simulink model "model_7dof&14dof"  (R2023b)
settings: Solver=FixedStepAuto  StartTime=0.0  StopTime=25  FixedStep=0.01  RelTol=1e-3  EnableMultiTasking=on
values from neighbouring files (symbols this model uses):
  A = 5    [unlinear_vehicle_Parameters.m]
  Bf = 1.725    [unlinear_vehicle_Parameters.m]
  Br = 1.750    (= 1.75)    [unlinear_vehicle_Parameters.m]
  Cd = 0.4    [unlinear_vehicle_Parameters.m]
  Cs_f = 4302    [unlinear_vehicle_Parameters.m]
  f = 0.01    [unlinear_vehicle_Parameters.m]
  g = 9.8    [Truck_simulate.m]    (also in unlinear_vehicle_Parameters.m)
  He = 0.45    [unlinear_vehicle_Parameters.m]
  hg = 0.781    [unlinear_vehicle_Parameters.m]
  Hp = 0.2    [unlinear_vehicle_Parameters.m]
  I_tire = 0.7    [unlinear_vehicle_Parameters.m]
  Ix = 423.3    [unlinear_vehicle_Parameters.m]
  Iy = 1762.5    [unlinear_vehicle_Parameters.m]
  Iz = 1762.5    [unlinear_vehicle_Parameters.m]
  ks_f = 189000    [unlinear_vehicle_Parameters.m]
  kw = 220000    [unlinear_vehicle_Parameters.m]
  L = 3.140    (= 3.14)    [unlinear_vehicle_Parameters.m]
  Lf = 1.330    (= 1.33)    [unlinear_vehicle_Parameters.m]
  Lr = 3.140 - 1.330    (= 1.81)    [unlinear_vehicle_Parameters.m]
  m = m_sprung + m_load + m_unsprung    (= 10505)    [Truck_simulate.m]    (also in unlinear_vehicle_Parameters.m = 1407.3)
  mb = 1128.5 + 000    (= 1128.5)    [unlinear_vehicle_Parameters.m]
  mw = 139.4 / 2    (= 69.7)    [unlinear_vehicle_Parameters.m]
  p = 1.206    [unlinear_vehicle_Parameters.m]
  r = 0.510    (= 0.51)    [Truck_simulate.m]    (also in unlinear_vehicle_Parameters.m = 0.287)
  vx0 = 5    [Truck_simulate.m]    (also in unlinear_vehicle_Parameters.m)
  vy0 = 0    [Truck_simulate.m]    (also in unlinear_vehicle_Parameters.m)
  w0 = vx0 / r    (= 9.80392156863)    [Truck_simulate.m]    (also in unlinear_vehicle_Parameters.m = 17.4216027875)
  wz0 = 0    [Truck_simulate.m]    (also in unlinear_vehicle_Parameters.m)
(part 2 of 2)

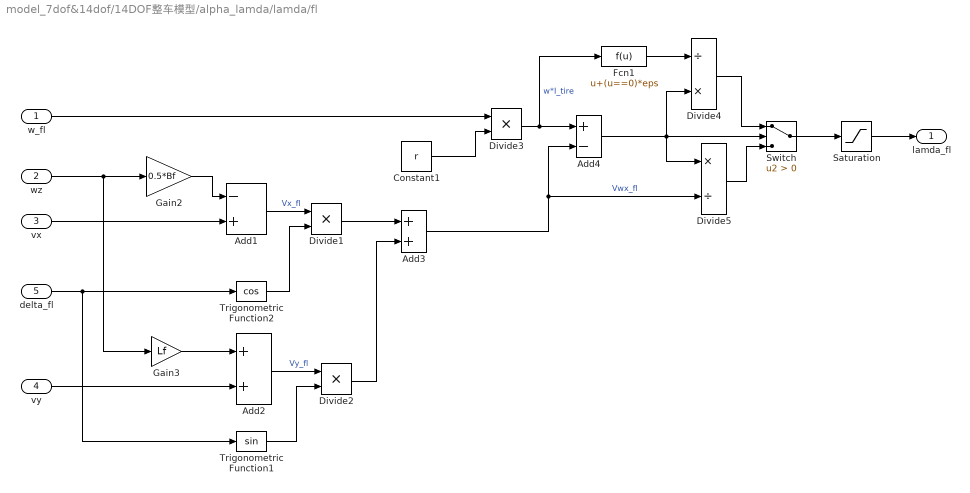
== system model_7dof&14dof/14DOF整车模型/alpha_lamda/lamda/fl ==
  w_fl : Inport
  wz : Inport  Port=2
  vx : Inport  Port=3
  vy : Inport  Port=4
  delta_fl : Inport  Port=5
  Add1 : Sum  Inputs=-+
  Add2 : Sum
  Add3 : Sum
  Add4 : Sum  Inputs=+-
  Constant1 : Constant  Value=r
  Divide1 : Product  Inputs=**
  Divide2 : Product  Inputs=**
  Divide3 : Product  Inputs=**
  Divide4 : Product  Inputs=/*
  Divide5 : Product  Inputs=*/
  Fcn1 : Fcn  Expr=u+(u==0)*eps
  Gain2 : Gain  Gain=0.5*Bf
  Gain3 : Gain  Gain=Lf
  Saturation : Saturate  UpperLimit=1  LowerLimit=-1
  Switch : Switch  Criteria=u2 > Threshold  SaturateOnIntegerOverflow=off  InputSameDT=off
  Trigonometric Function1 : Trigonometry
  Trigonometric Function2 : Trigonometry  Operator=cos
  lamda_fl : Outport
  wires:
  Saturation/1 -> lamda_fl/1
  Divide3/1 -> Fcn1/1, Add4/1  "w*I_tire"
  Constant1/1 -> Divide3/2
  w_fl/1 -> Divide3/1
  Divide2/1 -> Add3/2
  Divide1/1 -> Add3/1
  Trigonometric Function1/1 -> Divide2/2
  Add2/1 -> Divide2/1  "Vy_fl"
  Gain3/1 -> Add2/1
  vy/1 -> Add2/2
  Trigonometric Function2/1 -> Divide1/2
  delta_fl/1 -> Trigonometric Function1/1, Trigonometric Function2/1
  Add1/1 -> Divide1/1  "Vx_fl"
  wz/1 -> Gain2/1, Gain3/1
  Gain2/1 -> Add1/1
  vx/1 -> Add1/2
  Fcn1/1 -> Divide4/1
  Divide5/1 -> Switch/3
  Divide4/1 -> Switch/1
  Add4/1 -> Divide5/1, Divide4/2, Switch/2
  Add3/1 -> Divide5/2, Add4/2  "Vwx_fl"
  Switch/1 -> Saturation/1

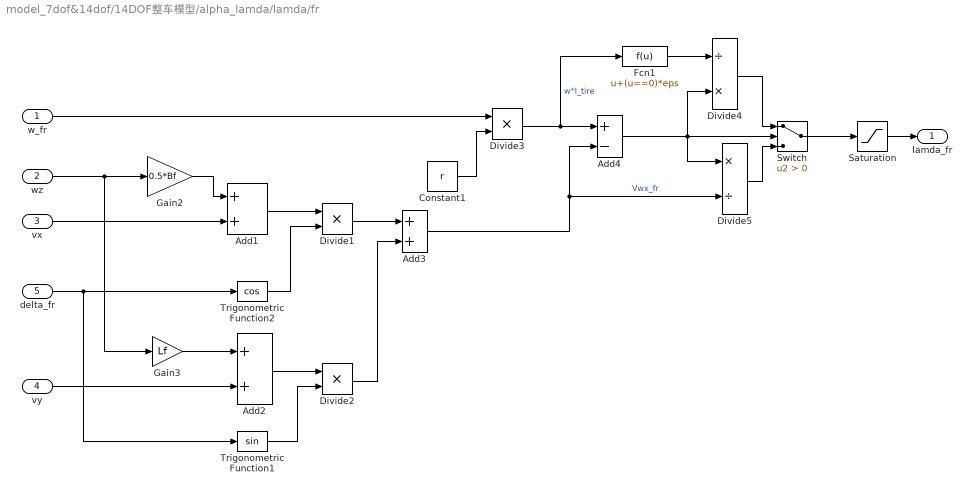
== system model_7dof&14dof/14DOF整车模型/alpha_lamda/lamda/fr ==
  w_fr : Inport
  wz : Inport  Port=2
  vx : Inport  Port=3
  vy : Inport  Port=4
  delta_fr : Inport  Port=5
  Add1 : Sum
  Add2 : Sum
  Add3 : Sum
  Add4 : Sum  Inputs=+-
  Constant1 : Constant  Value=r
  Divide1 : Product  Inputs=**
  Divide2 : Product  Inputs=**
  Divide3 : Product  Inputs=**
  Divide4 : Product  Inputs=/*
  Divide5 : Product  Inputs=*/
  Fcn1 : Fcn  Expr=u+(u==0)*eps
  Gain2 : Gain  Gain=0.5*Bf
  Gain3 : Gain  Gain=Lf
  Saturation : Saturate  UpperLimit=1  LowerLimit=-1
  Switch : Switch  Criteria=u2 > Threshold  SaturateOnIntegerOverflow=off  InputSameDT=off
  Trigonometric Function1 : Trigonometry
  Trigonometric Function2 : Trigonometry  Operator=cos
  lamda_fr : Outport
  wires:
  Switch/1 -> Saturation/1
  Add3/1 -> Add4/2, Divide5/2  "Vwx_fr"
  Add4/1 -> Switch/2, Divide4/2, Divide5/1
  Divide4/1 -> Switch/1
  Divide5/1 -> Switch/3
  Fcn1/1 -> Divide4/1
  Divide3/1 -> Add4/1, Fcn1/1  "w*I_tire"
  Constant1/1 -> Divide3/2
  w_fr/1 -> Divide3/1
  Divide2/1 -> Add3/2
  Divide1/1 -> Add3/1
  Trigonometric Function1/1 -> Divide2/2
  Add2/1 -> Divide2/1
  Gain3/1 -> Add2/1
  vy/1 -> Add2/2
  Trigonometric Function2/1 -> Divide1/2
  delta_fr/1 -> Trigonometric Function1/1, Trigonometric Function2/1
  Add1/1 -> Divide1/1
  wz/1 -> Gain2/1, Gain3/1
  Gain2/1 -> Add1/1
  vx/1 -> Add1/2
  Saturation/1 -> lamda_fr/1

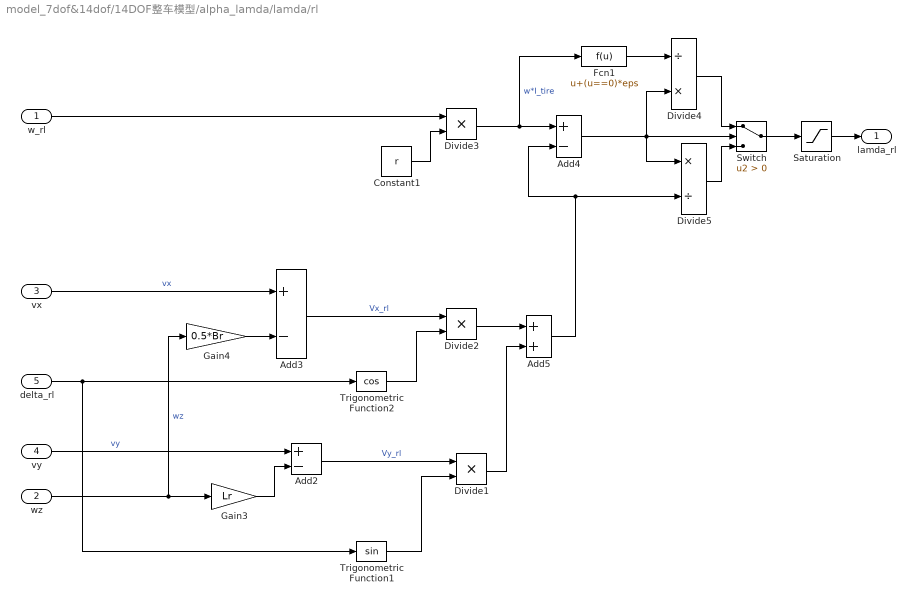
== system model_7dof&14dof/14DOF整车模型/alpha_lamda/lamda/rl ==
  w_rl : Inport
  wz : Inport  Port=2
  vx : Inport  Port=3
  vy : Inport  Port=4
  delta_rl : Inport  Port=5
  Add2 : Sum  Inputs=+-
  Add3 : Sum  Inputs=+-
  Add4 : Sum  Inputs=+-
  Add5 : Sum
  Constant1 : Constant  Value=r
  Divide1 : Product  Inputs=**
  Divide2 : Product  Inputs=**
  Divide3 : Product  Inputs=**
  Divide4 : Product  Inputs=/*
  Divide5 : Product  Inputs=*/
  Fcn1 : Fcn  Expr=u+(u==0)*eps
  Gain3 : Gain  Gain=Lr
  Gain4 : Gain  Gain=0.5*Br
  Saturation : Saturate  UpperLimit=1  LowerLimit=-1
  Switch : Switch  Criteria=u2 > Threshold  SaturateOnIntegerOverflow=off  InputSameDT=off
  Trigonometric Function1 : Trigonometry
  Trigonometric Function2 : Trigonometry  Operator=cos
  lamda_rl : Outport
  wires:
  Switch/1 -> Saturation/1
  Add4/1 -> Switch/2, Divide4/2, Divide5/1
  Divide4/1 -> Switch/1
  Divide5/1 -> Switch/3
  Fcn1/1 -> Divide4/1
  Divide3/1 -> Add4/1, Fcn1/1  "w*I_tire"
  Constant1/1 -> Divide3/2
  w_rl/1 -> Divide3/1
  Saturation/1 -> lamda_rl/1
  Gain4/1 -> Add3/2
  wz/1 -> Gain3/1, Gain4/1  "wz"
  vy/1 -> Add2/1  "vy"
  vx/1 -> Add3/1  "vx"
  Add3/1 -> Divide2/1  "Vx_rl"
  Add2/1 -> Divide1/1  "Vy_rl"
  Gain3/1 -> Add2/2
  delta_rl/1 -> Trigonometric Function1/1, Trigonometric Function2/1
  Trigonometric Function2/1 -> Divide2/2
  Divide2/1 -> Add5/1
  Trigonometric Function1/1 -> Divide1/2
  Divide1/1 -> Add5/2
  Add5/1 -> Add4/2, Divide5/2

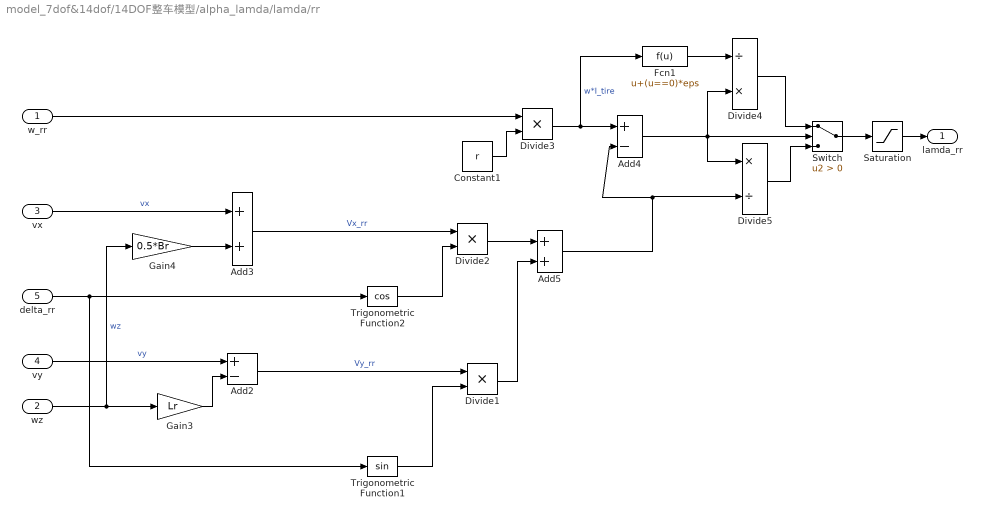
== system model_7dof&14dof/14DOF整车模型/alpha_lamda/lamda/rr ==
  w_rr : Inport
  wz : Inport  Port=2
  vx : Inport  Port=3
  vy : Inport  Port=4
  delta_rr : Inport  Port=5
  Add2 : Sum  Inputs=+-
  Add3 : Sum
  Add4 : Sum  Inputs=+-
  Add5 : Sum
  Constant1 : Constant  Value=r
  Divide1 : Product  Inputs=**
  Divide2 : Product  Inputs=**
  Divide3 : Product  Inputs=**
  Divide4 : Product  Inputs=/*
  Divide5 : Product  Inputs=*/
  Fcn1 : Fcn  Expr=u+(u==0)*eps
  Gain3 : Gain  Gain=Lr
  Gain4 : Gain  Gain=0.5*Br
  Saturation : Saturate  UpperLimit=1  LowerLimit=-1
  Switch : Switch  Criteria=u2 > Threshold  SaturateOnIntegerOverflow=off  InputSameDT=off
  Trigonometric Function1 : Trigonometry
  Trigonometric Function2 : Trigonometry  Operator=cos
  lamda_rr : Outport
  wires:
  Add4/1 -> Switch/2, Divide4/2, Divide5/1
  Divide4/1 -> Switch/1
  Divide5/1 -> Switch/3
  Fcn1/1 -> Divide4/1
  Divide3/1 -> Add4/1, Fcn1/1  "w*I_tire"
  w_rr/1 -> Divide3/1
  Constant1/1 -> Divide3/2
  Switch/1 -> Saturation/1
  Saturation/1 -> lamda_rr/1
  Gain4/1 -> Add3/2
  Gain3/1 -> Add2/2
  Add2/1 -> Divide1/1  "Vy_rr"
  Add3/1 -> Divide2/1  "Vx_rr"
  vx/1 -> Add3/1  "vx"
  vy/1 -> Add2/1  "vy"
  wz/1 -> Gain4/1, Gain3/1  "wz"
  Trigonometric Function2/1 -> Divide2/2
  Divide2/1 -> Add5/1
  Trigonometric Function1/1 -> Divide1/2
  Divide1/1 -> Add5/2
  delta_rr/1 -> Trigonometric Function1/1, Trigonometric Function2/1
  Add5/1 -> Add4/2, Divide5/2

== system model_7dof&14dof/7DOF整车模型/alpha_lamda/alpha/fl ==
  vx : Inport
  vy : Inport  Port=2
  wz : Inport  Port=3
  delta_fl : Inport  Port=4
  Add2 : Sum
  Add3 : Sum  Inputs=+-
  Add4 : Sum  Inputs=-+
  Divide : Product  Inputs=/*
  Gain3 : Gain  Gain=Lf
  Gain4 : Gain  Gain=0.5*Bf
  Trigonometric Function : Trigonometry  Operator=atan
  alpha_fl : Outport
  wires:
  wz/1 -> Gain3/1, Gain4/1
  Add4/1 -> alpha_fl/1
  vy/1 -> Add2/1
  delta_fl/1 -> Add4/2
  vx/1 -> Add3/1
  Trigonometric Function/1 -> Add4/1
  Divide/1 -> Trigonometric Function/1
  Add3/1 -> Divide/1
  Add2/1 -> Divide/2
  Gain4/1 -> Add3/2
  Gain3/1 -> Add2/2

== system model_7dof&14dof/7DOF整车模型/alpha_lamda/alpha/fr ==
  vx : Inport
  vy : Inport  Port=2
  wz : Inport  Port=3
  delta_fr : Inport  Port=4
  Add2 : Sum
  Add3 : Sum
  Add4 : Sum  Inputs=-+
  Divide : Product  Inputs=/*
  Gain3 : Gain  Gain=Lf
  Gain4 : Gain  Gain=0.5*Bf
  Trigonometric Function : Trigonometry  Operator=atan
  alpha_fr : Outport
  wires:
  Gain3/1 -> Add2/2
  Add2/1 -> Divide/2
  Add3/1 -> Divide/1
  Divide/1 -> Trigonometric Function/1
  Trigonometric Function/1 -> Add4/1
  vx/1 -> Add3/1
  delta_fr/1 -> Add4/2
  vy/1 -> Add2/1
  Add4/1 -> alpha_fr/1
  wz/1 -> Gain4/1, Gain3/1
  Gain4/1 -> Add3/2

== system model_7dof&14dof/7DOF整车模型/alpha_lamda/alpha/rl ==
  vx : Inport
  vy : Inport  Port=2
  wz : Inport  Port=3
  Add2 : Sum  Inputs=+-
  Add3 : Sum  Inputs=+-
  Divide : Product  Inputs=/*
  Gain1 : Gain  Gain=-1
  Gain3 : Gain  Gain=Lr
  Gain4 : Gain  Gain=0.5*Br
  Trigonometric Function : Trigonometry  Operator=atan
  alpha_rl : Outport
  wires:
  Gain3/1 -> Add2/2
  Add2/1 -> Divide/2
  Add3/1 -> Divide/1
  Divide/1 -> Trigonometric Function/1
  vx/1 -> Add3/1
  vy/1 -> Add2/1
  wz/1 -> Gain4/1, Gain3/1
  Trigonometric Function/1 -> Gain1/1
  Gain4/1 -> Add3/2
  Gain1/1 -> alpha_rl/1

== system model_7dof&14dof/7DOF整车模型/alpha_lamda/alpha/rr ==
  vx : Inport
  vy : Inport  Port=2
  wz : Inport  Port=3
  Add2 : Sum  Inputs=+-
  Add3 : Sum
  Divide : Product  Inputs=/*
  Gain2 : Gain  Gain=-1
  Gain3 : Gain  Gain=Lr
  Gain4 : Gain  Gain=0.5*Br
  Trigonometric Function : Trigonometry  Operator=atan
  alpha_rr : Outport
  wires:
  Trigonometric Function/1 -> Gain2/1
  wz/1 -> Gain3/1, Gain4/1
  vy/1 -> Add2/1
  vx/1 -> Add3/1
  Divide/1 -> Trigonometric Function/1
  Add3/1 -> Divide/1
  Add2/1 -> Divide/2
  Gain3/1 -> Add2/2
  Gain4/1 -> Add3/2
  Gain2/1 -> alpha_rr/1

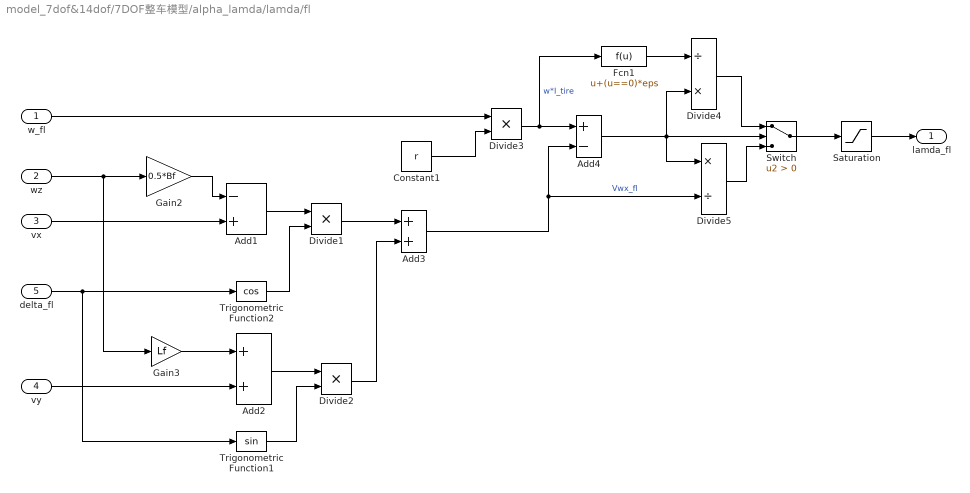
== system model_7dof&14dof/7DOF整车模型/alpha_lamda/lamda/fl ==
  w_fl : Inport
  wz : Inport  Port=2
  vx : Inport  Port=3
  vy : Inport  Port=4
  delta_fl : Inport  Port=5
  Add1 : Sum  Inputs=-+
  Add2 : Sum
  Add3 : Sum
  Add4 : Sum  Inputs=+-
  Constant1 : Constant  Value=r
  Divide1 : Product  Inputs=**
  Divide2 : Product  Inputs=**
  Divide3 : Product  Inputs=**
  Divide4 : Product  Inputs=/*
  Divide5 : Product  Inputs=*/
  Fcn1 : Fcn  Expr=u+(u==0)*eps
  Gain2 : Gain  Gain=0.5*Bf
  Gain3 : Gain  Gain=Lf
  Saturation : Saturate  UpperLimit=1  LowerLimit=-1
  Switch : Switch  Criteria=u2 > Threshold  SaturateOnIntegerOverflow=off  InputSameDT=off
  Trigonometric Function1 : Trigonometry
  Trigonometric Function2 : Trigonometry  Operator=cos
  lamda_fl : Outport
  wires:
  Switch/1 -> Saturation/1
  Add3/1 -> Add4/2, Divide5/2  "Vwx_fl"
  Add4/1 -> Switch/2, Divide4/2, Divide5/1
  Divide4/1 -> Switch/1
  Divide5/1 -> Switch/3
  Fcn1/1 -> Divide4/1
  vx/1 -> Add1/2
  Gain2/1 -> Add1/1
  wz/1 -> Gain3/1, Gain2/1
  Add1/1 -> Divide1/1
  delta_fl/1 -> Trigonometric Function2/1, Trigonometric Function1/1
  Trigonometric Function2/1 -> Divide1/2
  vy/1 -> Add2/2
  Gain3/1 -> Add2/1
  Add2/1 -> Divide2/1
  Trigonometric Function1/1 -> Divide2/2
  Divide1/1 -> Add3/1
  Divide2/1 -> Add3/2
  w_fl/1 -> Divide3/1
  Constant1/1 -> Divide3/2
  Divide3/1 -> Add4/1, Fcn1/1  "w*I_tire"
  Saturation/1 -> lamda_fl/1

== system model_7dof&14dof/7DOF整车模型/alpha_lamda/lamda/fr ==
  w_fr : Inport
  wz : Inport  Port=2
  vx : Inport  Port=3
  vy : Inport  Port=4
  delta_fr : Inport  Port=5
  Add1 : Sum
  Add2 : Sum
  Add3 : Sum
  Add4 : Sum  Inputs=+-
  Constant1 : Constant  Value=r
  Divide1 : Product  Inputs=**
  Divide2 : Product  Inputs=**
  Divide3 : Product  Inputs=**
  Divide4 : Product  Inputs=/*
  Divide5 : Product  Inputs=*/
  Fcn1 : Fcn  Expr=u+(u==0)*eps
  Gain2 : Gain  Gain=0.5*Bf
  Gain3 : Gain  Gain=Lf
  Saturation : Saturate  UpperLimit=1  LowerLimit=-1
  Switch : Switch  Criteria=u2 > Threshold  SaturateOnIntegerOverflow=off  InputSameDT=off
  Trigonometric Function1 : Trigonometry
  Trigonometric Function2 : Trigonometry  Operator=cos
  lamda_fr : Outport
  wires:
  Saturation/1 -> lamda_fr/1
  vx/1 -> Add1/2
  Gain2/1 -> Add1/1
  wz/1 -> Gain3/1, Gain2/1
  Add1/1 -> Divide1/1
  delta_fr/1 -> Trigonometric Function2/1, Trigonometric Function1/1
  Trigonometric Function2/1 -> Divide1/2
  vy/1 -> Add2/2
  Gain3/1 -> Add2/1
  Add2/1 -> Divide2/1
  Trigonometric Function1/1 -> Divide2/2
  Divide1/1 -> Add3/1
  Divide2/1 -> Add3/2
  w_fr/1 -> Divide3/1
  Constant1/1 -> Divide3/2
  Divide3/1 -> Fcn1/1, Add4/1  "w*I_tire"
  Fcn1/1 -> Divide4/1
  Divide5/1 -> Switch/3
  Divide4/1 -> Switch/1
  Add4/1 -> Divide5/1, Divide4/2, Switch/2
  Add3/1 -> Divide5/2, Add4/2  "Vwx_fr"
  Switch/1 -> Saturation/1

== system model_7dof&14dof/7DOF整车模型/alpha_lamda/lamda/rl ==
  w_rl : Inport
  wz : Inport  Port=2
  vx : Inport  Port=3
  Add1 : Sum  Inputs=-+
  Add4 : Sum  Inputs=+-
  Constant1 : Constant  Value=r
  Divide3 : Product  Inputs=**
  Divide4 : Product  Inputs=/*
  Divide5 : Product  Inputs=*/
  Fcn1 : Fcn  Expr=u+(u==0)*eps
  Gain2 : Gain  Gain=0.5*Br
  Saturation : Saturate  UpperLimit=1  LowerLimit=-1
  Switch : Switch  Criteria=u2 > Threshold  SaturateOnIntegerOverflow=off  InputSameDT=off
  lamda_rl : Outport
  wires:
  Saturation/1 -> lamda_rl/1
  vx/1 -> Add1/2
  Gain2/1 -> Add1/1
  wz/1 -> Gain2/1
  w_rl/1 -> Divide3/1
  Constant1/1 -> Divide3/2
  Divide3/1 -> Fcn1/1, Add4/1  "w*I_tire"
  Fcn1/1 -> Divide4/1
  Divide5/1 -> Switch/3
  Divide4/1 -> Switch/1
  Add4/1 -> Divide5/1, Divide4/2, Switch/2
  Add1/1 -> Divide5/2, Add4/2
  Switch/1 -> Saturation/1

== system model_7dof&14dof/7DOF整车模型/alpha_lamda/lamda/rr ==
  w_rr : Inport
  wz : Inport  Port=2
  vx : Inport  Port=3
  Add1 : Sum
  Add4 : Sum  Inputs=+-
  Constant1 : Constant  Value=r
  Divide3 : Product  Inputs=**
  Divide4 : Product  Inputs=/*
  Divide5 : Product  Inputs=*/
  Fcn1 : Fcn  Expr=u+(u==0)*eps
  Gain2 : Gain  Gain=0.5*Br
  Saturation : Saturate  UpperLimit=1  LowerLimit=-1
  Switch : Switch  Criteria=u2 > Threshold  SaturateOnIntegerOverflow=off  InputSameDT=off
  lamda_rr : Outport
  wires:
  Saturation/1 -> lamda_rr/1
  Switch/1 -> Saturation/1
  Constant1/1 -> Divide3/2
  w_rr/1 -> Divide3/1
  wz/1 -> Gain2/1
  Gain2/1 -> Add1/1
  vx/1 -> Add1/2
  Divide3/1 -> Fcn1/1, Add4/1  "w*I_tire"
  Fcn1/1 -> Divide4/1
  Divide5/1 -> Switch/3
  Divide4/1 -> Switch/1
  Add4/1 -> Divide5/1, Divide4/2, Switch/2
  Add1/1 -> Divide5/2, Add4/2  "Vwx_rr"

== matlab function model_7dof&14dof/7DOF整车模型/PAC2002/rl ==
  data: Fz input; Fx0 output; camber input; lamda input; alpha input; Fy0 output; Fx output; Fy output; Mz output; f input
function [Fx0,Fy0,Fx,Fy,Mz] = tire(Fz,camber,lamda,alpha,f)
if Fz>0
%Fz 轮胎垂向载荷 N
%camber 外倾角 rad？？？
%lamda 纵向滑移率
%alpha 车辆侧偏角 rad
alpha=tan(alpha);
camber=sin(camber);
Fz0=4607; %名义垂向载荷N
dfz=(Fz-Fz0)/Fz0;
%% Pure_Fx
%轮胎参数——纵向力
pcx1=1.65;
pdx1=1.3; pdx2=-0.15; pdx3=0;
pex1=0; pex2=0;pex3=0; pex4=0;
pkx1=20; pkx2=0; pkx3=0;
pvx1=0; pvx2=0;
phx1=0; phx2=0;
%pure_Fx 魔术公式
Cx=pcx1;
Shx=phx1+phx2*dfz;
lamda_x=lamda+Shx;
Dx=(pdx1+pdx2*dfz)*(1-pdx3*camber*camber)*Fz;
Ex=(pex1+pex2*dfz+pex3*dfz*dfz)*(1-pex4*sign(lamda_x));
Kx=Fz*(pkx1+pkx2*dfz)*exp(pkx3*dfz);
Bx=Kx/(Cx*Dx);
Svx=Fz*(pvx1+pvx2*dfz);
Fx0=Dx*sin(Cx*atan(Bx*lamda_x-Ex*(Bx*lamda_x-atan(Bx*lamda_x))))+Svx;
%% 联合工况纵向力Fx
%轮胎参数——纵向力
rbx1=20;rbx2=15;
rcx1=1;
rex1=0;rex2=0;
rhx1=0;
%纵向力加权函数
Bxa=rbx1*cos(atan(rbx2*lamda));
Cxa=rcx1;
Exa=rex1+rex2*dfz;
Shxa=rhx1;
alpha_s=alpha+Shxa;
Gxa=cos(Cxa*atan(Bxa*alpha_s-Exa*(Bxa*alpha_s-atan(Bxa*alpha_s))))/cos(Cxa*atan(Bxa*Shxa-Exa*(Bxa*Shxa-atan(Bxa*Shxa))));
Fx=Fx0*Gxa-f*Fz;



%% Pure_Fy
%轮胎参数——侧向力
pcy1=1.529245171;
pdy1=1.038581713; pdy2=-0.179464279; pdy3=-0.683745879;
pey1=-0.39012519; pey2=-0.611160145;pey3=-0.040677215; pey4=-14.95422065;
pky1=-26.056726760; pky2=2.106504624; pky3=0.499984439;
pvy1=0; pvy2=0;pvy3=0;pvy4=0;
phy1=0; phy2=0;phy3=0;
%pure_Fy 魔术公式
Cy=pcy1;
Shy=phy1+phy2*dfz+phy3*camber;
alpha_y=alpha+Shy;
uy=(pdy1+pdy2*dfz)*(1-pdy3*camber*camber);
Dy=uy*Fz;
Ey=(pey1+pey2*dfz)*(1-(pey3+pey4*camber)*sign(alpha_y));
Ky=pky1*Fz0*sin(2*atan(Fz/(pky2*Fz0)))*(1-pky3*abs(camber));
By=Ky/(Cy*Dy);
Svy=Fz*(pvy1+pvy2*dfz+(pvy3+pvy4*dfz)*camber);
Fy0=Dy*sin(Cy*atan(By*alpha_y-Ey*(By*alpha_y-atan(By*alpha_y))))+Svy;
%% 联合工况侧向力Fy
%轮胎参数——侧向力
rby1=10;rby2=10;rby3=-0.027856;
rcy1=1;
rey1=0;rey2=0;
rhy1=0;rhy2=0;
rvy1=0;rvy2=0;rvy3=0;rvy4=20;rvy5=2;rvy6=10;
%侧向力加权函数
Bya=rby1*cos(atan(rby2*(alpha-rby3)));
Cya=rcy1;
Eya=rey1+rey2*dfz;
Shya=rhy1+rhy2*dfz;
lamda_s=lamda+Shya;
Gya=cos(Cya*atan(Bya*lamda_s-Eya*(Bya*lamda_s-atan(Bya*lamda_s))))/cos(Cya*atan(Bya*Shya-Eya*(Bya*Shya-atan(Bya*Shya))));
%轮胎参数——侧向力
Svyr=uy*Fz*(rvy1+rvy2*dfz+rvy3*camber)*cos(atan(rvy4*alpha))*sin(rvy5*atan(rvy6*lamda));
Fy=Fy0*Gya+Svyr;

%% Pure_Mz
%轮胎参数——回正力矩
R0=0.357; %轮胎空载半径/m
qbz1=11.61018865;qbz2=-0.826853524;qbz3=-3.513951124;qbz4=0.063555994;qbz5=-1.014358836;
qcz1=1.064991884;
qdz1=0.091227598;qdz2=-0.001965108;qdz3=0.341001609;qdz4=-3.426482155;
qez1=-9.044014009;qez2=10;qez3=-19.59192084;qez4=0.156693082;qez5=-0.708977656;
%pure_Mz0 魔术公式
Ct=qcz1;
alpha_t=alpha;
Bt=(qbz1+qbz2*dfz+qbz3*dfz^2)*(1+qbz4*camber+qbz5*abs(camber));
Dt=Fz*(qdz1+qdz2*dfz)*(1+qdz3*camber+qdz4*camber^2)*R0/Fz0;
Et=(qez1+qez2*dfz+qez3*dfz^2)*(1+(qez4+qez5*camber)*((2/pi)*atan(Bt*Ct*alpha_t)));
t=Dt*cos(Ct*atan(Bt*alpha_t-Et*(Bt*alpha_t-atan(Bt*alpha_t))))*cos(alpha); %轮胎拖距
%轮胎参数——回正力矩
% qbz9=60;qbz10=1.177895045;
% qdz6=0.000688243;qdz7=0.002750679;qdz8=-0.303576739;qdz9=0.007781541;
%pure_Mz0 魔术公式
% Br=(qbz9+qbz10*By*Cy);
% Cr=1;
% Dr=Fz*(qdz6+qdz7*dfz+(qdz8+qdz9*dfz)*camber)*R0;
% alpha_r=alpha;
%Mzr=Dr*cos(Cr*atan(Br*alpha_r))*cos(alpha); %残余力矩
Mz=-t*Fy0;
else
    Fx0=0;
    Fy0=0;
    Fx=0;
    Fy=0;
    Mz=0;
end

== matlab function model_7dof&14dof/7DOF整车模型/PAC2002/rr ==
  data: Fz input; Fx0 output; camber input; lamda input; alpha input; Fy0 output; Fx output; Fy output; Mz output; f input
function [Fx0,Fy0,Fx,Fy,Mz] = tire(Fz,camber,lamda,alpha,f)
if Fz>0
%Fz 轮胎垂向载荷 N
%camber 外倾角 rad？？？
%lamda 纵向滑移率
%alpha 车辆侧偏角 rad
alpha=tan(alpha);
camber=sin(camber);
Fz0=4607; %名义垂向载荷N
dfz=(Fz-Fz0)/Fz0;
%% Pure_Fx
%轮胎参数——纵向力
pcx1=1.65;
pdx1=1.3; pdx2=-0.15; pdx3=0;
pex1=0; pex2=0;pex3=0; pex4=0;
pkx1=20; pkx2=0; pkx3=0;
pvx1=0; pvx2=0;
phx1=0; phx2=0;
%pure_Fx 魔术公式
Cx=pcx1;
Shx=phx1+phx2*dfz;
lamda_x=lamda+Shx;
Dx=(pdx1+pdx2*dfz)*(1-pdx3*camber*camber)*Fz;
Ex=(pex1+pex2*dfz+pex3*dfz*dfz)*(1-pex4*sign(lamda_x));
Kx=Fz*(pkx1+pkx2*dfz)*exp(pkx3*dfz);
Bx=Kx/(Cx*Dx);
Svx=Fz*(pvx1+pvx2*dfz);
Fx0=Dx*sin(Cx*atan(Bx*lamda_x-Ex*(Bx*lamda_x-atan(Bx*lamda_x))))+Svx;
%% 联合工况纵向力Fx
%轮胎参数——纵向力
rbx1=20;rbx2=15;
rcx1=1;
rex1=0;rex2=0;
rhx1=0;
%纵向力加权函数
Bxa=rbx1*cos(atan(rbx2*lamda));
Cxa=rcx1;
Exa=rex1+rex2*dfz;
Shxa=rhx1;
alpha_s=alpha+Shxa;
Gxa=cos(Cxa*atan(Bxa*alpha_s-Exa*(Bxa*alpha_s-atan(Bxa*alpha_s))))/cos(Cxa*atan(Bxa*Shxa-Exa*(Bxa*Shxa-atan(Bxa*Shxa))));
Fx=Fx0*Gxa-f*Fz;



%% Pure_Fy
%轮胎参数——侧向力
pcy1=1.529245171;
pdy1=1.038581713; pdy2=-0.179464279; pdy3=-0.683745879;
pey1=-0.39012519; pey2=-0.611160145;pey3=-0.040677215; pey4=-14.95422065;
pky1=-26.056726760; pky2=2.106504624; pky3=0.499984439;
pvy1=0; pvy2=0;pvy3=0;pvy4=0;
phy1=0; phy2=0;phy3=0;
%pure_Fy 魔术公式
Cy=pcy1;
Shy=phy1+phy2*dfz+phy3*camber;
alpha_y=alpha+Shy;
uy=(pdy1+pdy2*dfz)*(1-pdy3*camber*camber);
Dy=uy*Fz;
Ey=(pey1+pey2*dfz)*(1-(pey3+pey4*camber)*sign(alpha_y));
Ky=pky1*Fz0*sin(2*atan(Fz/(pky2*Fz0)))*(1-pky3*abs(camber));
By=Ky/(Cy*Dy);
Svy=Fz*(pvy1+pvy2*dfz+(pvy3+pvy4*dfz)*camber);
Fy0=Dy*sin(Cy*atan(By*alpha_y-Ey*(By*alpha_y-atan(By*alpha_y))))+Svy;
%% 联合工况侧向力Fy
%轮胎参数——侧向力
rby1=10;rby2=10;rby3=-0.027856;
rcy1=1;
rey1=0;rey2=0;
rhy1=0;rhy2=0;
rvy1=0;rvy2=0;rvy3=0;rvy4=20;rvy5=2;rvy6=10;
%侧向力加权函数
Bya=rby1*cos(atan(rby2*(alpha-rby3)));
Cya=rcy1;
Eya=rey1+rey2*dfz;
Shya=rhy1+rhy2*dfz;
lamda_s=lamda+Shya;
Gya=cos(Cya*atan(Bya*lamda_s-Eya*(Bya*lamda_s-atan(Bya*lamda_s))))/cos(Cya*atan(Bya*Shya-Eya*(Bya*Shya-atan(Bya*Shya))));
%轮胎参数——侧向力
Svyr=uy*Fz*(rvy1+rvy2*dfz+rvy3*camber)*cos(atan(rvy4*alpha))*sin(rvy5*atan(rvy6*lamda));
Fy=Fy0*Gya+Svyr;

%% Pure_Mz
%轮胎参数——回正力矩
R0=0.357; %轮胎空载半径/m
qbz1=11.61018865;qbz2=-0.826853524;qbz3=-3.513951124;qbz4=0.063555994;qbz5=-1.014358836;
qcz1=1.064991884;
qdz1=0.091227598;qdz2=-0.001965108;qdz3=0.341001609;qdz4=-3.426482155;
qez1=-9.044014009;qez2=10;qez3=-19.59192084;qez4=0.156693082;qez5=-0.708977656;
%pure_Mz0 魔术公式
Ct=qcz1;
alpha_t=alpha;
Bt=(qbz1+qbz2*dfz+qbz3*dfz^2)*(1+qbz4*camber+qbz5*abs(camber));
Dt=Fz*(qdz1+qdz2*dfz)*(1+qdz3*camber+qdz4*camber^2)*R0/Fz0;
Et=(qez1+qez2*dfz+qez3*dfz^2)*(1+(qez4+qez5*camber)*((2/pi)*atan(Bt*Ct*alpha_t)));
t=Dt*cos(Ct*atan(Bt*alpha_t-Et*(Bt*alpha_t-atan(Bt*alpha_t))))*cos(alpha); %轮胎拖距
%轮胎参数——回正力矩
% qbz9=60;qbz10=1.177895045;
% qdz6=0.000688243;qdz7=0.002750679;qdz8=-0.303576739;qdz9=0.007781541;
%pure_Mz0 魔术公式
% Br=(qbz9+qbz10*By*Cy);
% Cr=1;
% Dr=Fz*(qdz6+qdz7*dfz+(qdz8+qdz9*dfz)*camber)*R0;
% alpha_r=alpha;
%Mzr=Dr*cos(Cr*atan(Br*alpha_r))*cos(alpha); %残余力矩
Mz=-t*Fy0;
else
    Fx0=0;
    Fy0=0;
    Fx=0;
    Fy=0;
    Mz=0;
end

== matlab function model_7dof&14dof/14DOF整车模型/PAC2002/fr ==
  data: Fz input; Fx0 output; camber input; lamda input; alpha input; Fy0 output; Fx output; Fy output; Mz output; f input
function [Fx0,Fy0,Fx,Fy,Mz] = tire(Fz,camber,lamda,alpha,f)
if Fz>0
%Fz 轮胎垂向载荷 N
%camber 外倾角 rad？？？
%lamda 纵向滑移率
%alpha 车辆侧偏角 rad
alpha=tan(alpha);
camber=sin(camber);
Fz0=4100; %名义垂向载荷N
dfz=(Fz-Fz0)/Fz0;
%% Pure_Fx
%轮胎参数——纵向力
pcx1=1.62;
pdx1=1.035; pdx2=-0.0487; pdx3=-2.27;
pex1=0.5; pex2=-0.122;pex3=-0.063; pex4=0;
pkx1=19.4; pkx2=-0.13; pkx3=0.171;
pvx1=0; pvx2=0;
phx1=-0.0005; phx2=0.0000842;
%pure_Fx 魔术公式
Cx=pcx1;
Shx=phx1+phx2*dfz;
lamda_x=lamda+Shx;
Dx=(pdx1+pdx2*dfz)*(1-pdx3*camber*camber)*Fz;
Ex=(pex1+pex2*dfz+pex3*dfz*dfz)*(1-pex4*sign(lamda_x));
Kx=Fz*(pkx1+pkx2*dfz)*exp(pkx3*dfz);
Bx=Kx/(Cx*Dx);
Svx=Fz*(pvx1+pvx2*dfz);
Fx0=Dx*sin(Cx*atan(Bx*lamda_x-Ex*(Bx*lamda_x-atan(Bx*lamda_x))))+Svx;
%% 联合工况纵向力Fx
%轮胎参数——纵向力
rbx1=9.0;rbx2=-8.75;
rcx1=1.125;
rex1=0.078;rex2=-0.16;
rhx1=-0.03;
%纵向力加权函数
Bxa=rbx1*cos(atan(rbx2*lamda));
Cxa=rcx1;
Exa=rex1+rex2*dfz;
Shxa=rhx1;
alpha_s=alpha+Shxa;
Gxa=cos(Cxa*atan(Bxa*alpha_s-Exa*(Bxa*alpha_s-atan(Bxa*alpha_s))))/cos(Cxa*atan(Bxa*Shxa-Exa*(Bxa*Shxa-atan(Bxa*Shxa))));
Fx=Fx0*Gxa;



%% Pure_Fy
%轮胎参数——侧向力
pcy1=1.29;
pdy1=-0.9; pdy2=0.18; pdy3=-4.5;
pey1=-1.07; pey2=0.68;pey3=-0.63; pey4=-12.35;
pky1=-12.95; pky2=1.72; pky3=0.22;
pvy1=0.045; pvy2=-0.03;pvy3=-0.174;pvy4=-0.45;
phy1=0.0035; phy2=-0.003;phy3=0.045;
%pure_Fy 魔术公式
Cy=pcy1;
Shy=phy1+phy2*dfz+phy3*camber;
alpha_y=alpha+Shy;
uy=(pdy1+pdy2*dfz)*(1-pdy3*camber*camber);
Dy=uy*Fz;
Ey=(pey1+pey2*dfz)*(1-(pey3+pey4*camber)*sign(alpha_y));
Ky=pky1*Fz0*sin(2*atan(Fz/(pky2*Fz0)))*(1-pky3*abs(camber));
By=Ky/(Cy*Dy);
Svy=Fz*(pvy1+pvy2*dfz+(pvy3+pvy4*dfz)*camber);
Fy0=Dy*sin(Cy*atan(By*alpha_y-Ey*(By*alpha_y-atan(By*alpha_y))))+Svy;
%% 联合工况侧向力Fy
%轮胎参数——侧向力
rby1=6.38;rby2=7.95;rby3=-0.06;
rcy1=1.10;
rey1=0.23;rey2=0.41;
rhy1=0.0007;rhy2=0.024;
rvy1=0;rvy2=0;rvy3=0;rvy4=10;rvy5=1.95;rvy6=-50;
%侧向力加权函数
Bya=rby1*cos(atan(rby2*(alpha-rby3)));
Cya=rcy1;
Eya=rey1+rey2*dfz;
Shya=rhy1+rhy2*dfz;
lamda_s=lamda+Shya;
Gya=cos(Cya*atan(Bya*lamda_s-Eya*(Bya*lamda_s-atan(Bya*lamda_s))))/cos(Cya*atan(Bya*Shya-Eya*(Bya*Shya-atan(Bya*Shya))));
%轮胎参数——侧向力
Svyr=uy*Fz*(rvy1+rvy2*dfz+rvy3*camber)*cos(atan(rvy4*alpha))*sin(rvy5*atan(rvy6*lamda));
Fy=Fy0*Gya+Svyr;

%% Pure_Mz
%轮胎参数——回正力矩
R0=0.287; %轮胎空载半径/m
qbz1=8.37;qbz2=-2.92;qbz3=0.48;qbz4=-0.45;qbz5=-0.44;
qcz1=1.19;
qdz1=0.11;qdz2=-0.003;qdz3=-0.56;qdz4=8.40;
qez1=-2.9;qez2=-0.55;qez3=0;qez4=-0.13;qez5=-3.68;
%pure_Mz0 魔术公式
Ct=qcz1;
alpha_t=alpha;
Bt=(qbz1+qbz2*dfz+qbz3*dfz^2)*(1+qbz4*camber+qbz5*abs(camber));
Dt=Fz*(qdz1+qdz2*dfz)*(1+qdz3*camber+qdz4*camber^2)*R0/Fz0;
Et=(qez1+qez2*dfz+qez3*dfz^2)*(1+(qez4+qez5*camber)*((2/pi)*atan(Bt*Ct*alpha_t)));
t=Dt*cos(Ct*atan(Bt*alpha_t-Et*(Bt*alpha_t-atan(Bt*alpha_t))))*cos(alpha); %轮胎拖距
%轮胎参数——回正力矩
% qbz9=60;qbz10=1.177895045;
% qdz6=0.000688243;qdz7=0.002750679;qdz8=-0.303576739;qdz9=0.007781541;
%pure_Mz0 魔术公式
% Br=(qbz9+qbz10*By*Cy);
% Cr=1;
% Dr=Fz*(qdz6+qdz7*dfz+(qdz8+qdz9*dfz)*camber)*R0;
% alpha_r=alpha;
%Mzr=Dr*cos(Cr*atan(Br*alpha_r))*cos(alpha); %残余力矩
Mz=-t*Fy0;
else
    Fx0=0;
    Fy0=0;
    Fx=0;
    Fy=0;
    Mz=0;
end

== matlab function model_7dof&14dof/14DOF整车模型/PAC2002/rl ==
  data: Fz input; Fx0 output; camber input; lamda input; alpha input; Fy0 output; Fx output; Fy output; Mz output; f input
function [Fx0,Fy0,Fx,Fy,Mz] = tire(Fz,camber,lamda,alpha,f)
if Fz>0
%Fz 轮胎垂向载荷 N
%camber 外倾角 rad？？？
%lamda 纵向滑移率
%alpha 车辆侧偏角 rad
alpha=tan(alpha);
camber=sin(camber);
Fz0=4100; %名义垂向载荷N
dfz=(Fz-Fz0)/Fz0;
%% Pure_Fx
%轮胎参数——纵向力
pcx1=1.62;
pdx1=1.035; pdx2=-0.0487; pdx3=-2.27;
pex1=0.5; pex2=-0.122;pex3=-0.063; pex4=0;
pkx1=19.4; pkx2=-0.13; pkx3=0.171;
pvx1=0; pvx2=0;
phx1=-0.0005; phx2=0.0000842;
%pure_Fx 魔术公式
Cx=pcx1;
Shx=phx1+phx2*dfz;
lamda_x=lamda+Shx;
Dx=(pdx1+pdx2*dfz)*(1-pdx3*camber*camber)*Fz;
Ex=(pex1+pex2*dfz+pex3*dfz*dfz)*(1-pex4*sign(lamda_x));
Kx=Fz*(pkx1+pkx2*dfz)*exp(pkx3*dfz);
Bx=Kx/(Cx*Dx);
Svx=Fz*(pvx1+pvx2*dfz);
Fx0=Dx*sin(Cx*atan(Bx*lamda_x-Ex*(Bx*lamda_x-atan(Bx*lamda_x))))+Svx;
%% 联合工况纵向力Fx
%轮胎参数——纵向力
rbx1=9.0;rbx2=-8.75;
rcx1=1.125;
rex1=0.078;rex2=-0.16;
rhx1=-0.03;
%纵向力加权函数
Bxa=rbx1*cos(atan(rbx2*lamda));
Cxa=rcx1;
Exa=rex1+rex2*dfz;
Shxa=rhx1;
alpha_s=alpha+Shxa;
Gxa=cos(Cxa*atan(Bxa*alpha_s-Exa*(Bxa*alpha_s-atan(Bxa*alpha_s))))/cos(Cxa*atan(Bxa*Shxa-Exa*(Bxa*Shxa-atan(Bxa*Shxa))));
Fx=Fx0*Gxa;



%% Pure_Fy
%轮胎参数——侧向力
pcy1=1.29;
pdy1=-0.9; pdy2=0.18; pdy3=-4.5;
pey1=-1.07; pey2=0.68;pey3=-0.63; pey4=-12.35;
pky1=-12.95; pky2=1.72; pky3=0.22;
pvy1=0.045; pvy2=-0.03;pvy3=-0.174;pvy4=-0.45;
phy1=0.0035; phy2=-0.003;phy3=0.045;
%pure_Fy 魔术公式
Cy=pcy1;
Shy=phy1+phy2*dfz+phy3*camber;
alpha_y=alpha+Shy;
uy=(pdy1+pdy2*dfz)*(1-pdy3*camber*camber);
Dy=uy*Fz;
Ey=(pey1+pey2*dfz)*(1-(pey3+pey4*camber)*sign(alpha_y));
Ky=pky1*Fz0*sin(2*atan(Fz/(pky2*Fz0)))*(1-pky3*abs(camber));
By=Ky/(Cy*Dy);
Svy=Fz*(pvy1+pvy2*dfz+(pvy3+pvy4*dfz)*camber);
Fy0=Dy*sin(Cy*atan(By*alpha_y-Ey*(By*alpha_y-atan(By*alpha_y))))+Svy;
%% 联合工况侧向力Fy
%轮胎参数——侧向力
rby1=6.38;rby2=7.95;rby3=-0.06;
rcy1=1.10;
rey1=0.23;rey2=0.41;
rhy1=0.0007;rhy2=0.024;
rvy1=0;rvy2=0;rvy3=0;rvy4=10;rvy5=1.95;rvy6=-50;
%侧向力加权函数
Bya=rby1*cos(atan(rby2*(alpha-rby3)));
Cya=rcy1;
Eya=rey1+rey2*dfz;
Shya=rhy1+rhy2*dfz;
lamda_s=lamda+Shya;
Gya=cos(Cya*atan(Bya*lamda_s-Eya*(Bya*lamda_s-atan(Bya*lamda_s))))/cos(Cya*atan(Bya*Shya-Eya*(Bya*Shya-atan(Bya*Shya))));
%轮胎参数——侧向力
Svyr=uy*Fz*(rvy1+rvy2*dfz+rvy3*camber)*cos(atan(rvy4*alpha))*sin(rvy5*atan(rvy6*lamda));
Fy=Fy0*Gya+Svyr;

%% Pure_Mz
%轮胎参数——回正力矩
R0=0.287; %轮胎空载半径/m
qbz1=8.37;qbz2=-2.92;qbz3=0.48;qbz4=-0.45;qbz5=-0.44;
qcz1=1.19;
qdz1=0.11;qdz2=-0.003;qdz3=-0.56;qdz4=8.40;
qez1=-2.9;qez2=-0.55;qez3=0;qez4=-0.13;qez5=-3.68;
%pure_Mz0 魔术公式
Ct=qcz1;
alpha_t=alpha;
Bt=(qbz1+qbz2*dfz+qbz3*dfz^2)*(1+qbz4*camber+qbz5*abs(camber));
Dt=Fz*(qdz1+qdz2*dfz)*(1+qdz3*camber+qdz4*camber^2)*R0/Fz0;
Et=(qez1+qez2*dfz+qez3*dfz^2)*(1+(qez4+qez5*camber)*((2/pi)*atan(Bt*Ct*alpha_t)));
t=Dt*cos(Ct*atan(Bt*alpha_t-Et*(Bt*alpha_t-atan(Bt*alpha_t))))*cos(alpha); %轮胎拖距
%轮胎参数——回正力矩
% qbz9=60;qbz10=1.177895045;
% qdz6=0.000688243;qdz7=0.002750679;qdz8=-0.303576739;qdz9=0.007781541;
%pure_Mz0 魔术公式
% Br=(qbz9+qbz10*By*Cy);
% Cr=1;
% Dr=Fz*(qdz6+qdz7*dfz+(qdz8+qdz9*dfz)*camber)*R0;
% alpha_r=alpha;
%Mzr=Dr*cos(Cr*atan(Br*alpha_r))*cos(alpha); %残余力矩
Mz=-t*Fy0;
else
    Fx0=0;
    Fy0=0;
    Fx=0;
    Fy=0;
    Mz=0;
end

== matlab function model_7dof&14dof/14DOF整车模型/PAC2002/fl ==
  data: Fz input; Fx0 output; camber input; lamda input; alpha input; Fy0 output; Fx output; Fy output; Mz output; f input
function [Fx0,Fy0,Fx,Fy,Mz] = tire(Fz,camber,lamda,alpha,f)
if Fz>0
%Fz 轮胎垂向载荷 N
%camber 外倾角 rad
%lamda 纵向滑移率
%alpha 车辆侧偏角 rad
alpha=tan(alpha);
camber=sin(camber);
Fz0=4100; %名义垂向载荷N
dfz=(Fz-Fz0)/Fz0;
%% Pure_Fx
%轮胎参数——纵向力
pcx1=1.62;
pdx1=1.035; pdx2=-0.0487; pdx3=-2.27;
pex1=0.5; pex2=-0.122;pex3=-0.063; pex4=0;
pkx1=19.4; pkx2=-0.13; pkx3=0.171;
pvx1=0; pvx2=0;
phx1=-0.0005; phx2=0.0000842;
%pure_Fx 魔术公式
Cx=pcx1;
Shx=phx1+phx2*dfz;
lamda_x=lamda+Shx;
Dx=(pdx1+pdx2*dfz)*(1-pdx3*camber*camber)*Fz;
Ex=(pex1+pex2*dfz+pex3*dfz*dfz)*(1-pex4*sign(lamda_x));
Kx=Fz*(pkx1+pkx2*dfz)*exp(pkx3*dfz);
Bx=Kx/(Cx*Dx);
Svx=Fz*(pvx1+pvx2*dfz);
Fx0=Dx*sin(Cx*atan(Bx*lamda_x-Ex*(Bx*lamda_x-atan(Bx*lamda_x))))+Svx;
%% 联合工况纵向力Fx
%轮胎参数——纵向力
rbx1=9.0;rbx2=-8.75;
rcx1=1.125;
rex1=0.078;rex2=-0.16;
rhx1=-0.03;
%纵向力加权函数
Bxa=rbx1*cos(atan(rbx2*lamda));
Cxa=rcx1;
Exa=rex1+rex2*dfz;
Shxa=rhx1;
alpha_s=alpha+Shxa;
Gxa=cos(Cxa*atan(Bxa*alpha_s-Exa*(Bxa*alpha_s-atan(Bxa*alpha_s))))...
/cos(Cxa*atan(Bxa*Shxa-Exa*(Bxa*Shxa-atan(Bxa*Shxa))));
Fx=Fx0*Gxa;
%% Pure_Fy
%轮胎参数——侧向力
pcy1=1.29;
pdy1=-0.9; pdy2=0.18; pdy3=-4.5;
pey1=-1.07; pey2=0.68;pey3=-0.63; pey4=-12.35;
pky1=-12.95; pky2=1.72; pky3=0.22;
pvy1=0.045; pvy2=-0.03;pvy3=-0.174;pvy4=-0.45;
phy1=0.0035; phy2=-0.003;phy3=0.045;
%pure_Fy 魔术公式
Cy=pcy1;
Shy=phy1+phy2*dfz+phy3*camber;
alpha_y=alpha+Shy;
uy=(pdy1+pdy2*dfz)*(1-pdy3*camber*camber);
Dy=uy*Fz;
Ey=(pey1+pey2*dfz)*(1-(pey3+pey4*camber)*sign(alpha_y));
Ky=pky1*Fz0*sin(2*atan(Fz/(pky2*Fz0)))*(1-pky3*abs(camber));
By=Ky/(Cy*Dy);
Svy=Fz*(pvy1+pvy2*dfz+(pvy3+pvy4*dfz)*camber);
Fy0=Dy*sin(Cy*atan(By*alpha_y-Ey*(By*alpha_y-atan(By*alpha_y))))+Svy;
%% 联合工况侧向力Fy
%轮胎参数——侧向力
rby1=6.38;rby2=7.95;rby3=-0.06;
rcy1=1.10;
rey1=0.23;rey2=0.41;
rhy1=0.0007;rhy2=0.024;
rvy1=0;rvy2=0;rvy3=0;rvy4=10;rvy5=1.95;rvy6=-50;
%侧向力加权函数
Bya=rby1*cos(atan(rby2*(alpha-rby3)));
Cya=rcy1;
Eya=rey1+rey2*dfz;
Shya=rhy1+rhy2*dfz;
lamda_s=lamda+Shya;
Gya=cos(Cya*atan(Bya*lamda_s-Eya*(Bya*lamda_s-atan(Bya*lamda_s))))/cos(Cya*atan(Bya*Shya-Eya*(Bya*Shya-atan(Bya*Shya))));
%轮胎参数——侧向力
Svyr=uy*Fz*(rvy1+rvy2*dfz+rvy3*camber)*cos(atan(rvy4*alpha))*sin(rvy5*atan(rvy6*lamda));
Fy=Fy0*Gya+Svyr;

%% Pure_Mz
%轮胎参数——回正力矩
R0=0.287; %轮胎空载半径/m
qbz1=8.37;qbz2=-2.92;qbz3=0.48;qbz4=-0.45;qbz5=-0.44;
qcz1=1.19;
qdz1=0.11;qdz2=-0.003;qdz3=-0.56;qdz4=8.40;
qez1=-2.9;qez2=-0.55;qez3=0;qez4=-0.13;qez5=-3.68;
%pure_Mz0 魔术公式
Ct=qcz1;
alpha_t=alpha;
Bt=(qbz1+qbz2*dfz+qbz3*dfz^2)*(1+qbz4*camber+qbz5*abs(camber));
Dt=Fz*(qdz1+qdz2*dfz)*(1+qdz3*camber+qdz4*camber^2)*R0/Fz0;
Et=(qez1+qez2*dfz+qez3*dfz^2)*(1+(qez4+qez5*camber)*((2/pi)*atan(Bt*Ct*alpha_t)));
t=Dt*cos(Ct*atan(Bt*alpha_t-Et*(Bt*alpha_t-atan(Bt*alpha_t))))*cos(alpha); %轮胎拖距
%轮胎参数——回正力矩
% qbz9=60;qbz10=1.177895045;
% qdz6=0.000688243;qdz7=0.002750679;qdz8=-0.303576739;qdz9=0.007781541;
%pure_Mz0 魔术公式
% Br=(qbz9+qbz10*By*Cy);
% Cr=1;
% Dr=Fz*(qdz6+qdz7*dfz+(qdz8+qdz9*dfz)*camber)*R0;
% alpha_r=alpha;
%Mzr=Dr*cos(Cr*atan(Br*alpha_r))*cos(alpha); %残余力矩
Mz=-t*Fy0;
else
    Fx0=0;
    Fy0=0;
    Fx=0;
    Fy=0;
    Mz=0;
end

== matlab function model_7dof&14dof/14DOF整车模型/PAC2002/rr ==
  data: Fz input; Fx0 output; camber input; lamda input; alpha input; Fy0 output; Fx output; Fy output; Mz output; f input
function [Fx0,Fy0,Fx,Fy,Mz] = tire(Fz,camber,lamda,alpha,f)
if Fz>0
%Fz 轮胎垂向载荷 N
%camber 外倾角 rad？？？
%lamda 纵向滑移率
%alpha 车辆侧偏角 rad
alpha=tan(alpha);
camber=sin(camber);
Fz0=4100; %名义垂向载荷N
dfz=(Fz-Fz0)/Fz0;
%% Pure_Fx
%轮胎参数——纵向力
pcx1=1.62;
pdx1=1.035; pdx2=-0.0487; pdx3=-2.27;
pex1=0.5; pex2=-0.122;pex3=-0.063; pex4=0;
pkx1=19.4; pkx2=-0.13; pkx3=0.171;
pvx1=0; pvx2=0;
phx1=-0.0005; phx2=0.0000842;
%pure_Fx 魔术公式
Cx=pcx1;
Shx=phx1+phx2*dfz;
lamda_x=lamda+Shx;
Dx=(pdx1+pdx2*dfz)*(1-pdx3*camber*camber)*Fz;
Ex=(pex1+pex2*dfz+pex3*dfz*dfz)*(1-pex4*sign(lamda_x));
Kx=Fz*(pkx1+pkx2*dfz)*exp(pkx3*dfz);
Bx=Kx/(Cx*Dx);
Svx=Fz*(pvx1+pvx2*dfz);
Fx0=Dx*sin(Cx*atan(Bx*lamda_x-Ex*(Bx*lamda_x-atan(Bx*lamda_x))))+Svx;
%% 联合工况纵向力Fx
%轮胎参数——纵向力
rbx1=9.0;rbx2=-8.75;
rcx1=1.125;
rex1=0.078;rex2=-0.16;
rhx1=-0.03;
%纵向力加权函数
Bxa=rbx1*cos(atan(rbx2*lamda));
Cxa=rcx1;
Exa=rex1+rex2*dfz;
Shxa=rhx1;
alpha_s=alpha+Shxa;
Gxa=cos(Cxa*atan(Bxa*alpha_s-Exa*(Bxa*alpha_s-atan(Bxa*alpha_s))))/cos(Cxa*atan(Bxa*Shxa-Exa*(Bxa*Shxa-atan(Bxa*Shxa))));
Fx=Fx0*Gxa;



%% Pure_Fy
%轮胎参数——侧向力
pcy1=1.29;
pdy1=-0.9; pdy2=0.18; pdy3=-4.5;
pey1=-1.07; pey2=0.68;pey3=-0.63; pey4=-12.35;
pky1=-12.95; pky2=1.72; pky3=0.22;
pvy1=0.045; pvy2=-0.03;pvy3=-0.174;pvy4=-0.45;
phy1=0.0035; phy2=-0.003;phy3=0.045;
%pure_Fy 魔术公式
Cy=pcy1;
Shy=phy1+phy2*dfz+phy3*camber;
alpha_y=alpha+Shy;
uy=(pdy1+pdy2*dfz)*(1-pdy3*camber*camber);
Dy=uy*Fz;
Ey=(pey1+pey2*dfz)*(1-(pey3+pey4*camber)*sign(alpha_y));
Ky=pky1*Fz0*sin(2*atan(Fz/(pky2*Fz0)))*(1-pky3*abs(camber));
By=Ky/(Cy*Dy);
Svy=Fz*(pvy1+pvy2*dfz+(pvy3+pvy4*dfz)*camber);
Fy0=Dy*sin(Cy*atan(By*alpha_y-Ey*(By*alpha_y-atan(By*alpha_y))))+Svy;
%% 联合工况侧向力Fy
%轮胎参数——侧向力
rby1=6.38;rby2=7.95;rby3=-0.06;
rcy1=1.10;
rey1=0.23;rey2=0.41;
rhy1=0.0007;rhy2=0.024;
rvy1=0;rvy2=0;rvy3=0;rvy4=10;rvy5=1.95;rvy6=-50;
%侧向力加权函数
Bya=rby1*cos(atan(rby2*(alpha-rby3)));
Cya=rcy1;
Eya=rey1+rey2*dfz;
Shya=rhy1+rhy2*dfz;
lamda_s=lamda+Shya;
Gya=cos(Cya*atan(Bya*lamda_s-Eya*(Bya*lamda_s-atan(Bya*lamda_s))))/cos(Cya*atan(Bya*Shya-Eya*(Bya*Shya-atan(Bya*Shya))));
%轮胎参数——侧向力
Svyr=uy*Fz*(rvy1+rvy2*dfz+rvy3*camber)*cos(atan(rvy4*alpha))*sin(rvy5*atan(rvy6*lamda));
Fy=Fy0*Gya+Svyr;

%% Pure_Mz
%轮胎参数——回正力矩
R0=0.287; %轮胎空载半径/m
qbz1=8.37;qbz2=-2.92;qbz3=0.48;qbz4=-0.45;qbz5=-0.44;
qcz1=1.19;
qdz1=0.11;qdz2=-0.003;qdz3=-0.56;qdz4=8.40;
qez1=-2.9;qez2=-0.55;qez3=0;qez4=-0.13;qez5=-3.68;
%pure_Mz0 魔术公式
Ct=qcz1;
alpha_t=alpha;
Bt=(qbz1+qbz2*dfz+qbz3*dfz^2)*(1+qbz4*camber+qbz5*abs(camber));
Dt=Fz*(qdz1+qdz2*dfz)*(1+qdz3*camber+qdz4*camber^2)*R0/Fz0;
Et=(qez1+qez2*dfz+qez3*dfz^2)*(1+(qez4+qez5*camber)*((2/pi)*atan(Bt*Ct*alpha_t)));
t=Dt*cos(Ct*atan(Bt*alpha_t-Et*(Bt*alpha_t-atan(Bt*alpha_t))))*cos(alpha); %轮胎拖距
%轮胎参数——回正力矩
% qbz9=60;qbz10=1.177895045;
% qdz6=0.000688243;qdz7=0.002750679;qdz8=-0.303576739;qdz9=0.007781541;
%pure_Mz0 魔术公式
% Br=(qbz9+qbz10*By*Cy);
% Cr=1;
% Dr=Fz*(qdz6+qdz7*dfz+(qdz8+qdz9*dfz)*camber)*R0;
% alpha_r=alpha;
%Mzr=Dr*cos(Cr*atan(Br*alpha_r))*cos(alpha); %残余力矩
Mz=-t*Fy0;
else
    Fx0=0;
    Fy0=0;
    Fx=0;
    Fy=0;
    Mz=0;
end

== matlab function model_7dof&14dof/7DOF整车模型/PAC2002/fl ==
  data: Fz input; Fx0 output; camber input; lamda input; alpha input; Fy0 output; Fx output; Fy output; Mz output; f input
function [Fx0,Fy0,Fx,Fy,Mz] = tire(Fz,camber,lamda,alpha,f)
if Fz>0
%Fz 轮胎垂向载荷 N
%camber 外倾角 rad？？？
%lamda 纵向滑移率
%alpha 车辆侧偏角 rad
alpha=tan(alpha);
camber=sin(camber);
Fz0=4607; %名义垂向载荷N
dfz=(Fz-Fz0)/Fz0;
%% Pure_Fx
%轮胎参数——纵向力
pcx1=1.65;
pdx1=1.3; pdx2=-0.15; pdx3=0;
pex1=0; pex2=0;pex3=0; pex4=0;
pkx1=20; pkx2=0; pkx3=0;
pvx1=0; pvx2=0;
phx1=0; phx2=0;
%pure_Fx 魔术公式
Cx=pcx1;
Shx=phx1+phx2*dfz;
lamda_x=lamda+Shx;
Dx=(pdx1+pdx2*dfz)*(1-pdx3*camber*camber)*Fz;
Ex=(pex1+pex2*dfz+pex3*dfz*dfz)*(1-pex4*sign(lamda_x));
Kx=Fz*(pkx1+pkx2*dfz)*exp(pkx3*dfz);
Bx=Kx/(Cx*Dx);
Svx=Fz*(pvx1+pvx2*dfz);
Fx0=Dx*sin(Cx*atan(Bx*lamda_x-Ex*(Bx*lamda_x-atan(Bx*lamda_x))))+Svx;
%% 联合工况纵向力Fx
%轮胎参数——纵向力
rbx1=20;rbx2=15;
rcx1=1;
rex1=0;rex2=0;
rhx1=0;
%纵向力加权函数
Bxa=rbx1*cos(atan(rbx2*lamda));
Cxa=rcx1;
Exa=rex1+rex2*dfz;
Shxa=rhx1;
alpha_s=alpha+Shxa;
Gxa=cos(Cxa*atan(Bxa*alpha_s-Exa*(Bxa*alpha_s-atan(Bxa*alpha_s))))/cos(Cxa*atan(Bxa*Shxa-Exa*(Bxa*Shxa-atan(Bxa*Shxa))));
Fx=Fx0*Gxa-Fz*f;



%% Pure_Fy
%轮胎参数——侧向力
pcy1=1.529245171;
pdy1=1.038581713; pdy2=-0.179464279; pdy3=-0.683745879;
pey1=-0.39012519; pey2=-0.611160145;pey3=-0.040677215; pey4=-14.95422065;
pky1=-26.056726760; pky2=2.106504624; pky3=0.499984439;
pvy1=0; pvy2=0;pvy3=0;pvy4=0;
phy1=0; phy2=0;phy3=0;
%pure_Fy 魔术公式
Cy=pcy1;
Shy=phy1+phy2*dfz+phy3*camber;
alpha_y=alpha+Shy;
uy=(pdy1+pdy2*dfz)*(1-pdy3*camber*camber);
Dy=uy*Fz;
Ey=(pey1+pey2*dfz)*(1-(pey3+pey4*camber)*sign(alpha_y));
Ky=pky1*Fz0*sin(2*atan(Fz/(pky2*Fz0)))*(1-pky3*abs(camber));
By=Ky/(Cy*Dy);
Svy=Fz*(pvy1+pvy2*dfz+(pvy3+pvy4*dfz)*camber);
Fy0=Dy*sin(Cy*atan(By*alpha_y-Ey*(By*alpha_y-atan(By*alpha_y))))+Svy;
%% 联合工况侧向力Fy
%轮胎参数——侧向力
rby1=10;rby2=10;rby3=-0.027856;
rcy1=1;
rey1=0;rey2=0;
rhy1=0;rhy2=0;
rvy1=0;rvy2=0;rvy3=0;rvy4=20;rvy5=2;rvy6=10;
%侧向力加权函数
Bya=rby1*cos(atan(rby2*(alpha-rby3)));
Cya=rcy1;
Eya=rey1+rey2*dfz;
Shya=rhy1+rhy2*dfz;
lamda_s=lamda+Shya;
Gya=cos(Cya*atan(Bya*lamda_s-Eya*(Bya*lamda_s-atan(Bya*lamda_s))))/cos(Cya*atan(Bya*Shya-Eya*(Bya*Shya-atan(Bya*Shya))));
%轮胎参数——侧向力
Svyr=uy*Fz*(rvy1+rvy2*dfz+rvy3*camber)*cos(atan(rvy4*alpha))*sin(rvy5*atan(rvy6*lamda));
Fy=Fy0*Gya+Svyr;

%% Pure_Mz
%轮胎参数——回正力矩
R0=0.357; %轮胎空载半径/m
qbz1=11.61018865;qbz2=-0.826853524;qbz3=-3.513951124;qbz4=0.063555994;qbz5=-1.014358836;
qcz1=1.064991884;
qdz1=0.091227598;qdz2=-0.001965108;qdz3=0.341001609;qdz4=-3.426482155;
qez1=-9.044014009;qez2=10;qez3=-19.59192084;qez4=0.156693082;qez5=-0.708977656;
%pure_Mz0 魔术公式
Ct=qcz1;
alpha_t=alpha;
Bt=(qbz1+qbz2*dfz+qbz3*dfz^2)*(1+qbz4*camber+qbz5*abs(camber));
Dt=Fz*(qdz1+qdz2*dfz)*(1+qdz3*camber+qdz4*camber^2)*R0/Fz0;
Et=(qez1+qez2*dfz+qez3*dfz^2)*(1+(qez4+qez5*camber)*((2/pi)*atan(Bt*Ct*alpha_t)));
t=Dt*cos(Ct*atan(Bt*alpha_t-Et*(Bt*alpha_t-atan(Bt*alpha_t))))*cos(alpha); %轮胎拖距
%轮胎参数——回正力矩
% qbz9=60;qbz10=1.177895045;
% qdz6=0.000688243;qdz7=0.002750679;qdz8=-0.303576739;qdz9=0.007781541;
%pure_Mz0 魔术公式
% Br=(qbz9+qbz10*By*Cy);
% Cr=1;
% Dr=Fz*(qdz6+qdz7*dfz+(qdz8+qdz9*dfz)*camber)*R0;
% alpha_r=alpha;
%Mzr=Dr*cos(Cr*atan(Br*alpha_r))*cos(alpha); %残余力矩
Mz=-t*Fy0;
else
    Fx0=0;
    Fy0=0;
    Fx=0;
    Fy=0;
    Mz=0;
end

== matlab function model_7dof&14dof/7DOF整车模型/PAC2002/fr ==
  data: Fz input; Fx0 output; camber input; lamda input; alpha input; Fy0 output; Fx output; Fy output; Mz output; f input
function [Fx0,Fy0,Fx,Fy,Mz] = tire(Fz,camber,lamda,alpha,f)
if Fz>0
%Fz 轮胎垂向载荷 N
%camber 外倾角 rad？？？
%lamda 纵向滑移率
%alpha 车辆侧偏角 rad
alpha=tan(alpha);
camber=sin(camber);
Fz0=4607; %名义垂向载荷N
dfz=(Fz-Fz0)/Fz0;
%% Pure_Fx
%轮胎参数——纵向力
pcx1=1.65;
pdx1=1.3; pdx2=-0.15; pdx3=0;
pex1=0; pex2=0;pex3=0; pex4=0;
pkx1=20; pkx2=0; pkx3=0;
pvx1=0; pvx2=0;
phx1=0; phx2=0;
%pure_Fx 魔术公式
Cx=pcx1;
Shx=phx1+phx2*dfz;
lamda_x=lamda+Shx;
Dx=(pdx1+pdx2*dfz)*(1-pdx3*camber*camber)*Fz;
Ex=(pex1+pex2*dfz+pex3*dfz*dfz)*(1-pex4*sign(lamda_x));
Kx=Fz*(pkx1+pkx2*dfz)*exp(pkx3*dfz);
Bx=Kx/(Cx*Dx);
Svx=Fz*(pvx1+pvx2*dfz);
Fx0=Dx*sin(Cx*atan(Bx*lamda_x-Ex*(Bx*lamda_x-atan(Bx*lamda_x))))+Svx;
%% 联合工况纵向力Fx
%轮胎参数——纵向力
rbx1=20;rbx2=15;
rcx1=1;
rex1=0;rex2=0;
rhx1=0;
%纵向力加权函数
Bxa=rbx1*cos(atan(rbx2*lamda));
Cxa=rcx1;
Exa=rex1+rex2*dfz;
Shxa=rhx1;
alpha_s=alpha+Shxa;
Gxa=cos(Cxa*atan(Bxa*alpha_s-Exa*(Bxa*alpha_s-atan(Bxa*alpha_s))))/cos(Cxa*atan(Bxa*Shxa-Exa*(Bxa*Shxa-atan(Bxa*Shxa))));
Fx=Fx0*Gxa-f*Fz;



%% Pure_Fy
%轮胎参数——侧向力
pcy1=1.529245171;
pdy1=1.038581713; pdy2=-0.179464279; pdy3=-0.683745879;
pey1=-0.39012519; pey2=-0.611160145;pey3=-0.040677215; pey4=-14.95422065;
pky1=-26.056726760; pky2=2.106504624; pky3=0.499984439;
pvy1=0; pvy2=0;pvy3=0;pvy4=0;
phy1=0; phy2=0;phy3=0;
%pure_Fy 魔术公式
Cy=pcy1;
Shy=phy1+phy2*dfz+phy3*camber;
alpha_y=alpha+Shy;
uy=(pdy1+pdy2*dfz)*(1-pdy3*camber*camber);
Dy=uy*Fz;
Ey=(pey1+pey2*dfz)*(1-(pey3+pey4*camber)*sign(alpha_y));
Ky=pky1*Fz0*sin(2*atan(Fz/(pky2*Fz0)))*(1-pky3*abs(camber));
By=Ky/(Cy*Dy);
Svy=Fz*(pvy1+pvy2*dfz+(pvy3+pvy4*dfz)*camber);
Fy0=Dy*sin(Cy*atan(By*alpha_y-Ey*(By*alpha_y-atan(By*alpha_y))))+Svy;
%% 联合工况侧向力Fy
%轮胎参数——侧向力
rby1=10;rby2=10;rby3=-0.027856;
rcy1=1;
rey1=0;rey2=0;
rhy1=0;rhy2=0;
rvy1=0;rvy2=0;rvy3=0;rvy4=20;rvy5=2;rvy6=10;
%侧向力加权函数
Bya=rby1*cos(atan(rby2*(alpha-rby3)));
Cya=rcy1;
Eya=rey1+rey2*dfz;
Shya=rhy1+rhy2*dfz;
lamda_s=lamda+Shya;
Gya=cos(Cya*atan(Bya*lamda_s-Eya*(Bya*lamda_s-atan(Bya*lamda_s))))/cos(Cya*atan(Bya*Shya-Eya*(Bya*Shya-atan(Bya*Shya))));
%轮胎参数——侧向力
Svyr=uy*Fz*(rvy1+rvy2*dfz+rvy3*camber)*cos(atan(rvy4*alpha))*sin(rvy5*atan(rvy6*lamda));
Fy=Fy0*Gya+Svyr;

%% Pure_Mz
%轮胎参数——回正力矩
R0=0.357; %轮胎空载半径/m
qbz1=11.61018865;qbz2=-0.826853524;qbz3=-3.513951124;qbz4=0.063555994;qbz5=-1.014358836;
qcz1=1.064991884;
qdz1=0.091227598;qdz2=-0.001965108;qdz3=0.341001609;qdz4=-3.426482155;
qez1=-9.044014009;qez2=10;qez3=-19.59192084;qez4=0.156693082;qez5=-0.708977656;
%pure_Mz0 魔术公式
Ct=qcz1;
alpha_t=alpha;
Bt=(qbz1+qbz2*dfz+qbz3*dfz^2)*(1+qbz4*camber+qbz5*abs(camber));
Dt=Fz*(qdz1+qdz2*dfz)*(1+qdz3*camber+qdz4*camber^2)*R0/Fz0;
Et=(qez1+qez2*dfz+qez3*dfz^2)*(1+(qez4+qez5*camber)*((2/pi)*atan(Bt*Ct*alpha_t)));
t=Dt*cos(Ct*atan(Bt*alpha_t-Et*(Bt*alpha_t-atan(Bt*alpha_t))))*cos(alpha); %轮胎拖距
%轮胎参数——回正力矩
% qbz9=60;qbz10=1.177895045;
% qdz6=0.000688243;qdz7=0.002750679;qdz8=-0.303576739;qdz9=0.007781541;
%pure_Mz0 魔术公式
% Br=(qbz9+qbz10*By*Cy);
% Cr=1;
% Dr=Fz*(qdz6+qdz7*dfz+(qdz8+qdz9*dfz)*camber)*R0;
% alpha_r=alpha;
%Mzr=Dr*cos(Cr*atan(Br*alpha_r))*cos(alpha); %残余力矩
Mz=-t*Fy0;
else
    Fx0=0;
    Fy0=0;
    Fx=0;
    Fy=0;
    Mz=0;
end
